simulink model "General_MPC_with_Cubic_Ls_Correction_Pose"  (R2026b)
settings: Solver=FixedStepDiscrete  StopTime=60
model workspace (MAT data in the model file):
  Velocity = 27.7777777778
  Wheel_Base = 2.866
values from neighbouring files (symbols this model uses):
  Point_Init = 0.0    [Path.sldd]
  Pose_Correction_Init = 0    [Pose_Correction.sldd]
  Pose_Init = 0.0    [MPC_Main_Dictionary.sldd]
  Reference_Path_Init = 0.0    [Path.sldd]
  Station_Calc_Init = 0.0    [Path.sldd]
  Trajectory_Init = 0.0    [Path.sldd]
  Vehicle_Cmd_Init = 0.0    [Vehicle_Controller.sldd]
libraries: simulink_extras x1
settings Model: DataDictionary=MPC_Main_Dictionary.sldd  Creator=손상민  LastModifiedBy=손상민
settings OptimizationCC: DefaultParameterBehavior=Inlined  DifferentSizesBufferReuse=on  EfficientTunableParamExpr=on  EnhancedBackFolding=on  OptimizationCustomize=off  OptimizeBlockOrder=speed  PassReuseOutputArgsAs=Individual arguments  RemoveInternalMemoryZeroInit=on  RemoveRootLevelIOMemoryZeroInit=on
settings DebuggingCC: ParameterTunabilityLossMsg=error
settings RTWCC: DataTypeReplacement=CDataTypesFixedWidth  Description=Embedded Coder  SystemTargetFile=ert.tlc  TemplateMakefile=ert_default_tmf
settings CodeAppCC: ForceParamTrailComments=on  IgnoreCustomStorageClasses=off  InsertBlockDesc=on  OperatorAnnotations=on  SFDataObjDesc=on  SimulinkDataObjDesc=on
settings ERTTargetCC: CombineSignalStateStructs=on  GenerateSampleERTMain=on  MaxIdInt16=INT16_MAX  MaxIdInt32=INT32_MAX  MaxIdInt64=INT64_MAX  MaxIdInt8=INT8_MAX  MaxIdUint16=UINT16_MAX  MaxIdUint32=UINT32_MAX  MaxIdUint64=UINT64_MAX  MaxIdUint8=UINT8_MAX  MinIdInt16=INT16_MIN  MinIdInt32=INT32_MIN  MinIdInt64=INT64_MIN  MinIdInt8=INT8_MIN

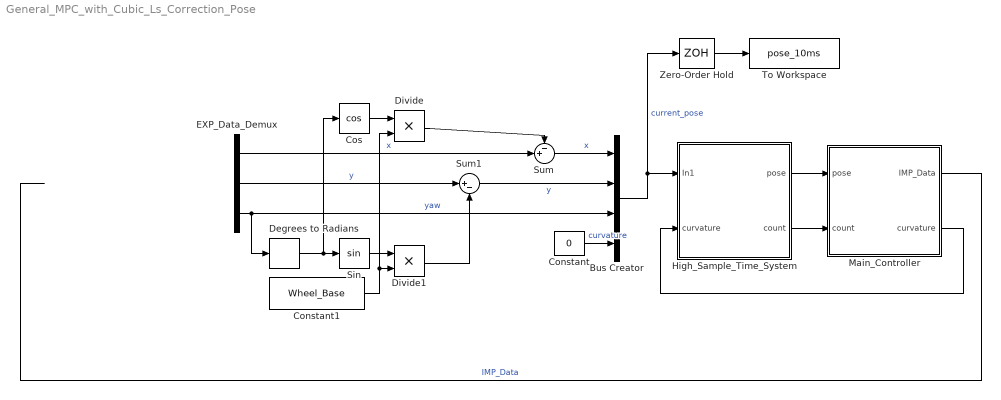
== system General_MPC_with_Cubic_Ls_Correction_Pose ==
  Bus Creator : BusCreator  Inputs=4  OutDataTypeStr=Bus: Point  NonVirtualBus=on
  Constant : Constant  Value=0
  Constant1 : Constant  Value=Wheel_Base
  Cos : Trigonometry  Operator=cos
  Degrees to Radians : simulink_extras/Transformations/Degrees to Radians
  Divide : Product  Inputs=**
  Divide1 : Product  Inputs=**
  EXP_Data_Demux : Demux  Outputs=3
  High_Sample_Time_System : Subsystem  TreatAsAtomicUnit=on  SystemSampleTime=0.1
  Main_Controller : Subsystem  TreatAsAtomicUnit=on  SystemSampleTime=0.02
  Sin : Trigonometry
  Sum : Sum  Inputs=-+|
  Sum1 : Sum  Inputs=|+-
  To Workspace : ToWorkspace  VariableName=pose_10ms  SaveFormat=Timeseries  SampleTime=-1
  Zero-Order Hold : ZeroOrderHold  SampleTime=0.01
  wires:
  Main_Controller/1(IMP_Data) -> ?  "IMP_Data"
  Zero-Order Hold/1 -> To Workspace/1
  High_Sample_Time_System/1(pose) -> Main_Controller/1(pose)
  High_Sample_Time_System/2(count) -> Main_Controller/2(count)
  EXP_Data_Demux/1 -> Sum/2  "x"
  EXP_Data_Demux/2 -> Sum1/1  "y"
  EXP_Data_Demux/3 -> Degrees to Radians/1, Bus Creator/3  "yaw"
  Constant/1 -> Bus Creator/4  "curvature"
  ? -> EXP_Data_Demux/1  "EXP_Data"
  Degrees to Radians/1 -> Cos/1, Sin/1
  Constant1/1 -> Divide/2, Divide1/2
  Cos/1 -> Divide/1
  Sin/1 -> Divide1/1
  Divide1/1 -> Sum1/2
  Sum1/1 -> Bus Creator/2  "y"
  Divide/1 -> Sum/1
  Sum/1 -> Bus Creator/1  "x"
  Bus Creator/1 -> Zero-Order Hold/1, High_Sample_Time_System/1(In1)  "current_pose"
  Main_Controller/2(curvature) -> High_Sample_Time_System/2(curvature)

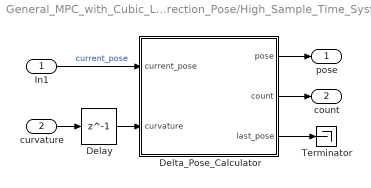
== system General_MPC_with_Cubic_Ls_Correction_Pose/High_Sample_Time_System ==
  In1 : Inport
  curvature : Inport  Port=2
  Delay : Delay  DelayLength=1  InputProcessing=Columns as channels (frame based)
  Delta_Pose_Calculator : Stateflow chart  TreatAsAtomicUnit=on
  Terminator : Terminator
  pose : Outport  OutDataTypeStr=Bus: Point
  count : Outport  Port=2  OutDataTypeStr=uint32
  wires:
  In1/1 -> Delta_Pose_Calculator/1(current_pose)  "current_pose"
  Delta_Pose_Calculator/3(last_pose) -> Terminator/1
  Delta_Pose_Calculator/2(count) -> count/1
  Delta_Pose_Calculator/1(pose) -> pose/1
  curvature/1 -> Delay/1
  Delay/1 -> Delta_Pose_Calculator/2(curvature)

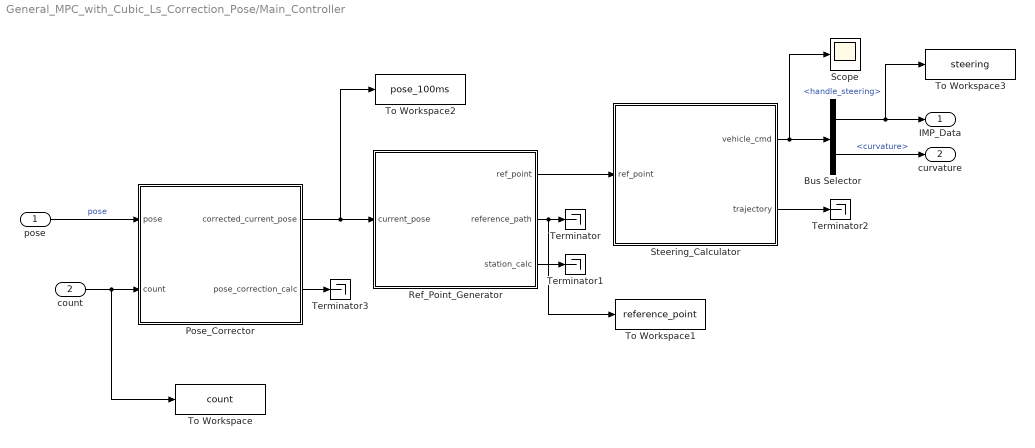
== system General_MPC_with_Cubic_Ls_Correction_Pose/Main_Controller ==
  pose : Inport  OutDataTypeStr=Bus: Point
  count : Inport  Port=2  OutDataTypeStr=uint32
  Bus Selector : BusSelector  OutputSignals=handle_steering,curvature
  Pose_Corrector : Stateflow chart  TreatAsAtomicUnit=on
  Ref_Point_Generator : Stateflow chart  TreatAsAtomicUnit=on
  Scope : Scope
      settings: ActiveDisplayYMinimum=-65.96053155183364  ActiveDisplayYMaximum=44.846225949844211
  Steering_Calculator : Stateflow chart  TreatAsAtomicUnit=on
  Terminator{,1..3} (4 alike) : Terminator
  To Workspace : ToWorkspace  VariableName=count  SaveFormat=Timeseries  SampleTime=-1
  To Workspace1 : ToWorkspace  VariableName=reference_point  SaveFormat=Timeseries  SampleTime=-1
  To Workspace2 : ToWorkspace  VariableName=pose_100ms  SaveFormat=Timeseries  SampleTime=-1
  To Workspace3 : ToWorkspace  VariableName=steering  SaveFormat=Timeseries  SampleTime=-1
  IMP_Data : Outport
  curvature : Outport  Port=2
  wires:
  pose/1 -> Pose_Corrector/1(pose)  "pose"
  Ref_Point_Generator/2(reference_path) -> To Workspace1/1, Terminator/1
  Ref_Point_Generator/1(ref_point) -> Steering_Calculator/1(ref_point)
  Steering_Calculator/1(vehicle_cmd) -> Scope/1, Bus Selector/1
  Ref_Point_Generator/3(station_calc) -> Terminator1/1
  Bus Selector/1 -> To Workspace3/1, IMP_Data/1  "<handle_steering>"
  Bus Selector/2 -> curvature/1  "<curvature>"
  Steering_Calculator/2(trajectory) -> Terminator2/1
  Pose_Corrector/1(corrected_current_pose) -> To Workspace2/1, Ref_Point_Generator/1(current_pose)
  count/1 -> To Workspace/1, Pose_Corrector/2(count)
  Pose_Corrector/2(pose_correction_calc) -> Terminator3/1

== matlab function General_MPC_with_Cubic_Ls_Correction_Pose/Main_Controller/Steering_Calculator ==
  data: out_para function_output Bus: Point size=201; out_para function_output Bus: Vehicle_Cmd size=1; out_para function_output double size=1; ref_point input Bus: Point size=1; vehicle_cmd output Bus: Vehicle_Cmd size=1 =Vehicle_Cmd_Init; trajectory output Bus: Point size=201 =Trajectory_Init
function out_para = Generate_Trajectory

out_para = trajectory;

sampleTime = 0.1;
wheelbase = 2.866;
velocity = 30/3.6;
steering = deg2rad(vehicle_cmd.steering);

predictionHorizon = 15;

xTarget = ref_point.x;
yTarget = ref_point.y;
headingTarget = wrap_to_pi_local(ref_point.yaw);
curvatureTarget = ref_point.curvature;

heading0 = 0.0;
curvature0 = tan(steering) / wheelbase;

pointSpacing = sampleTime * abs(velocity);
pointCount = predictionHorizon + 1;

chordLength = hypot(xTarget, yTarget);

if chordLength <= 1.0e-6 || pointSpacing <= 1.0e-12
    for i = 1:pointCount
        out_para(i).x = 0.0;
        out_para(i).y = 0.0;
        out_para(i).yaw = 0.0;
        out_para(i).curvature = curvature0;
    end
    return
end

tangent0 = [cos(heading0), sin(heading0)];
tangent1 = [cos(headingTarget), sin(headingTarget)];

normal0 = [-sin(heading0), cos(heading0)];
normal1 = [-sin(headingTarget), cos(headingTarget)];

velocity0 = chordLength * tangent0;
velocity1 = chordLength * tangent1;

acceleration0 = chordLength^2 * curvature0 * normal0;
acceleration1 = chordLength^2 * curvatureTarget * normal1;

boundaryMatrix = [ ...
    1, 0, 0,  0,  0,  0;
    0, 1, 0,  0,  0,  0;
    0, 0, 2,  0,  0,  0;
    1, 1, 1,  1,  1,  1;
    0, 1, 2,  3,  4,  5;
    0, 0, 2,  6, 12, 20];

boundaryValues = [ ...
    0.0, 0.0;
    velocity0;
    acceleration0;
    xTarget, yTarget;
    velocity1;
    acceleration1];

coeff = boundaryMatrix \ boundaryValues;

denseCount = 10001;
uDense = linspace(0.0, 1.0, denseCount).';

[denseX, denseY, ~, ~, ~, ~] = ...
    evaluate_polynomial(coeff, uDense);

denseArc = [0.0; cumsum(hypot(diff(denseX), diff(denseY)))];
totalLength = denseArc(end);

requestedArc = (0:predictionHorizon).' * pointSpacing;
requestedArc = min(requestedArc, totalLength);

u = invert_arc_length(denseArc, uDense, requestedArc);

[x, y, dx, dy, ddx, ddy] = ...
    evaluate_polynomial(coeff, u);

speedSquared = dx.^2 + dy.^2;
speedSquared = max(speedSquared, 1.0e-12);

yaw = atan2(dy, dx);

curvature = ...
    (dx .* ddy - dy .* ddx) ./ ...
    (speedSquared .^ 1.5);

for i = 1:pointCount
    out_para(i).x = x(i);
    out_para(i).y = y(i);
    out_para(i).yaw = yaw(i);
    out_para(i).curvature = curvature(i);
end

end


function uQuery = invert_arc_length(arcValues, uValues, queryValues)

queryCount = numel(queryValues);
arcCount = numel(arcValues);

uQuery = zeros(queryCount, 1);

searchIndex = 1;

for i = 1:queryCount

    queryArc = queryValues(i);

    if queryArc <= arcValues(1)

        uQuery(i) = uValues(1);

    elseif queryArc >= arcValues(arcCount)

        uQuery(i) = uValues(arcCount);

    else

        while searchIndex < arcCount && ...
                arcValues(searchIndex + 1) < queryArc

            searchIndex = searchIndex + 1;

        end

        lowerIndex = searchIndex;
        upperIndex = lowerIndex + 1;

        while upperIndex <= arcCount && ...
                arcValues(upperIndex) <= arcValues(lowerIndex)

            upperIndex = upperIndex + 1;

        end

        if upperIndex > arcCount

            uQuery(i) = uValues(lowerIndex);

        else

            arcInterval = ...
                arcValues(upperIndex) - arcValues(lowerIndex);

            ratio = ...
                (queryArc - arcValues(lowerIndex)) / arcInterval;

            ratio = min(max(ratio, 0.0), 1.0);

            uQuery(i) = ...
                uValues(lowerIndex) + ...
                ratio * (uValues(upperIndex) - uValues(lowerIndex));

        end
    end
end

end


function [x, y, dx, dy, ddx, ddy] = evaluate_polynomial(coeff, u)

basis0 = [ ...
    ones(size(u)), ...
    u, ...
    u.^2, ...
    u.^3, ...
    u.^4, ...
    u.^5];

basis1 = [ ...
    zeros(size(u)), ...
    ones(size(u)), ...
    2*u, ...
    3*u.^2, ...
    4*u.^3, ...
    5*u.^4];

basis2 = [ ...
    zeros(size(u)), ...
    zeros(size(u)), ...
    2*ones(size(u)), ...
    6*u, ...
    12*u.^2, ...
    20*u.^3];

position = basis0 * coeff;
firstDerivative = basis1 * coeff;
secondDerivative = basis2 * coeff;

x = position(:, 1);
y = position(:, 2);

dx = firstDerivative(:, 1);
dy = firstDerivative(:, 2);

ddx = secondDerivative(:, 1);
ddy = secondDerivative(:, 2);

end


function angle = wrap_to_pi_local(angle)

angle = mod(angle + pi, 2*pi) - pi;

end

== matlab function General_MPC_with_Cubic_Ls_Correction_Pose/Main_Controller/Steering_Calculator ==
function out_para = MPC

out_para = vehicle_cmd;

sampleTime = 0.1;
wheelbase = 2.866;

predictionHorizon = double(15);
controlHorizon = double(10);

wheelSteering = deg2rad(vehicle_cmd.steering);
targetSpeed = 30/3.6;

traj = zeros(4, predictionHorizon + 1);

for index = 1:predictionHorizon + 1
    traj(1,index) = trajectory(index).x;
    traj(2,index) = trajectory(index).y;
    traj(3,index) = trajectory(index).yaw;
    traj(4,index) = trajectory(index).curvature;
end

R = 500 * eye(controlHorizon);
F = 200 * eye(controlHorizon);
Q = kron(eye(predictionHorizon), diag([100 500 500]));

steerMax = deg2rad(35);
duMax = deg2rad(5);

W = tril(ones(controlHorizon));

Aineq = [W; -W];

bineq = [ ...
    steerMax * ones(controlHorizon,1) - wheelSteering;
    steerMax * ones(controlHorizon,1) + wheelSteering];

A_k = [ ...
    1 0 -targetSpeed * sin(traj(3,2)) * sampleTime;
    0 1  targetSpeed * cos(traj(3,2)) * sampleTime;
    0 0  1];

B_k = [ ...
    0;
    0;
    targetSpeed * sampleTime / wheelbase];

Abar_k = zeros(4);
Abar_k(1:3,1:3) = A_k;
Abar_k(1:3,4) = B_k;
Abar_k(4,4) = 1;

Bbar_k = [B_k; 1];

cbar = [eye(3), zeros(3,1)];

Psi_k = zeros(3 * predictionHorizon, 4);

for row = 1:predictionHorizon
    Psi_k(3*row-2:3*row,:) = ...
        cbar * (Abar_k^row);
end

Theta_k = zeros(3 * predictionHorizon, controlHorizon);

for row = 1:predictionHorizon
    for col = 1:controlHorizon

        powerValue = row - col;

        if powerValue >= 0
            Theta_k(3*row-2:3*row,col) = ...
                cbar * (Abar_k^powerValue) * Bbar_k;
        end

    end
end

Pi_k = zeros(3 * predictionHorizon, 4 * predictionHorizon);

for row = 1:predictionHorizon
    for col = 1:predictionHorizon

        powerValue = row - col;

        if powerValue >= 0
            Pi_k(3*row-2:3*row,4*col-3:4*col) = ...
                cbar * (Abar_k^powerValue);
        end

    end
end

steeringRef = atan(wheelbase * traj(4,:));

X_ref = [ ...
    traj(1:3,:);
    steeringRef];

G_k = zeros(4 * predictionHorizon, 1);

for row = 1:predictionHorizon

    duRef = steeringRef(row+1) - steeringRef(row);

    G_k(4*row-3:4*row) = ...
        X_ref(:,row+1) ...
        - Abar_k * X_ref(:,row) ...
        - Bbar_k * duRef;

end

Y_ref = reshape( ...
    traj(1:3,2:predictionHorizon+1), ...
    [], 1);

X0 = [ ...
    traj(1:3,1);
    wheelSteering];

E_k = ...
    Psi_k * X0 ...
    + Pi_k * G_k ...
    - Y_ref;

U_ref = steeringRef(2:controlHorizon+1).';

EU_k = ...
    ones(controlHorizon,1) * wheelSteering ...
    - U_ref;

S_k = ...
    2 * E_k.' * Q * Theta_k ...
    + 2 * EU_k.' * F * W;

H_k = 2 * ( ...
    Theta_k.' * Q * Theta_k ...
    + R ...
    + W.' * F * W);

H_k = 0.5 * (H_k + H_k.');

options = optimoptions( ...
    'quadprog', ...
    'Algorithm', 'active-set', ...
    'Display', 'off');

lb = -duMax * ones(controlHorizon,1);
ub =  duMax * ones(controlHorizon,1);

x0 = zeros(controlHorizon,1);

dU = quadprog( ...
    H_k, ...
    S_k.', ...
    Aineq, ...
    bineq, ...
    [], ...
    [], ...
    lb, ...
    ub, ...
    x0, ...
    options);

if isempty(dU)
    outWheelSteering = wheelSteering;
else
    outWheelSteering = wheelSteering + dU(1);
end

out_para.steering = rad2deg(outWheelSteering);
out_para.curvature = tan(outWheelSteering) / wheelbase;

end

== matlab function General_MPC_with_Cubic_Ls_Correction_Pose/Main_Controller/Steering_Calculator ==
function out_para = Calc_Handle_Steering

equivalentSteerDeg = [ ...
    -38.0000000015 -37.5537097659 -37.1100763419 -36.6690267064 -36.2304905472 -35.7944001026 ...
    -35.3606900619 -34.9292974092 -34.5001613191 -34.0732230402 -33.6484257893 -33.2257146793 ...
    -32.8050365911 -32.3863401170 -31.9695754559 -31.5546943618 -31.1416500661 -30.7303971963 ...
    -30.3208917313 -29.9130909189 -29.5069532444 -29.1024383621 -28.6995070462 -28.2981211430 ...
    -27.8982435354 -27.4998380812 -27.1028695774 -26.7073037505 -26.3131071606 -25.9202472249 ...
    -25.5286921549 -25.1384109184 -24.7493732347 -24.3615495211 -23.9749108816 -23.5894290638 ...
    -23.2050764567 -22.8218260419 -22.4396513910 -22.0585266399 -21.6784264440 -21.2993259988 ...
    -20.9212009824 -20.5440275610 -20.1677823626 -19.7924424606 -19.4179853631 -19.0443889805 ...
    -18.6716316310 -18.2996920094 -17.9285491937 -17.5581826079 -17.1885720119 -16.8196975175 ...
    -16.4515395418 -16.0840788091 -15.7172963351 -15.3511734516 -14.9856917222 -14.6208329945 ...
    -14.2565793874 -13.8929132418 -13.5298171372 -13.1672739009 -12.8052665504 -12.4437783367 ...
    -12.0827926977 -11.7222932796 -11.3622638965 -11.0026885634 -10.6435514521 -10.2848369165 ...
    -9.9265294385 -9.5686136760 -9.2110744293 -8.8538966284 -8.4970653414 -8.1405657596 ...
    -7.7843831967 -7.4285030781 -7.0729109402 -6.7175924190 -6.3625332509 -6.0077192620 ...
    -5.6531363648 -5.2987705549 -4.9446079016 -4.5906345476 -4.2368366983 -3.8832006231 ...
    -3.5297126453 -3.1763591407 -2.8231265306 -2.4700012785 -2.1169698838 -1.7640188790 ...
    -1.4111348234 -1.0583043010 -0.7055139116 -0.3527502699 0.0000000000 0.3527502699 ...
    0.7055139116 1.0583043010 1.4111348234 1.7640188790 2.1169698838 2.4700012785 ...
    2.8231265306 3.1763591407 3.5297126453 3.8832006231 4.2368366983 4.5906345476 ...
    4.9446079016 5.2987705549 5.6531363648 6.0077192620 6.3625332509 6.7175924190 ...
    7.0729109402 7.4285030781 7.7843831967 8.1405657596 8.4970653414 8.8538966284 ...
    9.2110744293 9.5686136760 9.9265294385 10.2848369165 10.6435514521 11.0026885634 ...
    11.3622638965 11.7222932796 12.0827926977 12.4437783367 12.8052665504 13.1672739009 ...
    13.5298171372 13.8929132418 14.2565793874 14.6208329945 14.9856917222 15.3511734516 ...
    15.7172963351 16.0840788091 16.4515395418 16.8196975175 17.1885720119 17.5581826079 ...
    17.9285491937 18.2996920094 18.6716316310 19.0443889805 19.4179853631 19.7924424606 ...
    20.1677823626 20.5440275610 20.9212009824 21.2993259988 21.6784264440 22.0585266399 ...
    22.4396513910 22.8218260419 23.2050764567 23.5894290638 23.9749108816 24.3615495211 ...
    24.7493732347 25.1384109184 25.5286921549 25.9202472249 26.3131071606 26.7073037505 ...
    27.1028695774 27.4998380812 27.8982435354 28.2981211430 28.6995070462 29.1024383621 ...
    29.5069532444 29.9130909189 30.3208917313 30.7303971963 31.1416500661 31.5546943618 ...
    31.9695754559 32.3863401170 32.8050365911 33.2257146793 33.6484257893 34.0732230402 ...
    34.5001613191 34.9292974092 35.3606900619 35.7944001026 36.2304905472 36.6690267064 ...
    37.1100763419 37.5537097659 38.0000000015
    ].';

rackMap = (-90.0:0.9:90.0).';

wheelSteeringDeg = vehicle_cmd.steering;

rackDisplacement = interp1(equivalentSteerDeg, rackMap, wheelSteeringDeg, 'linear');
out_para = rackDisplacement * 360.0 / 56.25;

end

== matlab function General_MPC_with_Cubic_Ls_Correction_Pose/High_Sample_Time_System/Delta_Pose_Calculator ==
  data: out_para function_output; pose output Bus: Point size=5 =Pose_Init; current_pose input Bus: Point size=1; count output uint32 size=1 =0; last_pose output Bus: Point size=1 =Point_Init; curvature input double size=1
function out_para = Calc_Delta_Pose 

out_para = pose;

index = mod(count,5) + 1;

out_para(index) = current_pose;
out_para(index).curvature = curvature;

== matlab function General_MPC_with_Cubic_Ls_Correction_Pose/Main_Controller/Ref_Point_Generator ==
  data: out_para function_output Bus: Reference_Path size=1; out_para function_output Bus: Station_Calc size=1; out_para function_output Bus: Point size=1; ref_point output Bus: Point size=1 =Point_Init; reference_path output Bus: Reference_Path size=1 =Reference_Path_Init; current_pose input Bus: Point size=1; station_calc output Bus: Station_Calc size=1 =Station_Calc_Init
function out_para = Map_Generator 

out_para = reference_path;

ds = 0.1;

x_data = [70 75 80 85 90 95 100 105 110 115 120 125 130 135 140 145];
y_data = [0 0.2 1.1 2.4 3.3 3.5 3.5 3.5 3.5 3.5 3.5 3.3 2.4 1.1 0.2 0];

pp = spline(x_data, [0 y_data 0]);

x_temp = linspace(0, 500, 10000);
y_temp = zeros(size(x_temp));

idx = (x_temp >= 70) & (x_temp <= 145);
y_temp(idx) = ppval(pp, x_temp(idx));

s_temp = [0 cumsum(hypot(diff(x_temp), diff(y_temp)))];

station = 0:ds:5007;

x = interp1(s_temp, x_temp, station, 'pchip');
y = interp1(s_temp, y_temp, station, 'pchip');

dx_ds = gradient(x, station);
dy_ds = gradient(y, station);

yaw = unwrap(atan2(dy_ds, dx_ds));

ddx_ds2 = gradient(dx_ds, station);
ddy_ds2 = gradient(dy_ds, station);

curvature = (dx_ds .* ddy_ds2 - dy_ds .* ddx_ds2) ./ ...
    (dx_ds.^2 + dy_ds.^2).^(3/2);

N = length(x);

for i = 1:N
    out_para.points(i).x = x(i);
    out_para.points(i).y = y(i);
    out_para.points(i).yaw = yaw(i);
    out_para.points(i).curvature = curvature(i);
end

out_para.length = uint32(N);

== matlab function General_MPC_with_Cubic_Ls_Correction_Pose/Main_Controller/Ref_Point_Generator ==
function out_para = Calc_Station 

out_para = station_calc;

min_dist = inf;
start_idx = double(out_para.station_index);

if out_para.predictive_length == 0

    % initialize
    for i = 1:reference_path.length
        dx = reference_path.points(i).x - current_pose.x;
        dy = reference_path.points(i).y - current_pose.y;

        dist = dx * dx + dy * dy;

        if dist < min_dist
            min_dist = dist;
            out_para.station_index = uint32(i);
        end
    end

else

    for i = 1:out_para.predictive_length
        dx = out_para.predictive_station(i).x - current_pose.x;
        dy = out_para.predictive_station(i).y - current_pose.y;

        dist = dx * dx + dy * dy;

        if dist < min_dist
            min_dist = dist;
            out_para.station_index = uint32(start_idx + i - 1);
        end
    end

end

N_ref = double(reference_path.length);
start_idx = double(out_para.station_index);

N_pred = min(50, N_ref - start_idx + 1);

for i = 1:N_pred
    idx = start_idx + i - 1;

    out_para.predictive_station(i).x = reference_path.points(idx).x;
    out_para.predictive_station(i).y = reference_path.points(idx).y;
    out_para.predictive_station(i).yaw = reference_path.points(idx).yaw;
    out_para.predictive_station(i).curvature = reference_path.points(idx).curvature;
end

out_para.predictive_length = uint32(N_pred);

== matlab function General_MPC_with_Cubic_Ls_Correction_Pose/Main_Controller/Ref_Point_Generator ==
function out_para = Calc_Ref_Point 

out_para = ref_point;

ds = 0.1;
velocity = 30/3.6;
preview_second = 1.5;
 
preview_distance = velocity * preview_second;

preview_index = double(station_calc.station_index) + round(preview_distance / ds);
preview_index = min(preview_index, double(reference_path.length));

ref = reference_path.points(preview_index);

dx = ref.x - current_pose.x;
dy = ref.y - current_pose.y;

yaw = deg2rad(current_pose.yaw);
c = cos(yaw);
s = sin(yaw);

out_para.x =  c * dx + s * dy;
out_para.y = -s * dx + c * dy;
out_para.yaw = atan2(sin(ref.yaw - yaw), cos(ref.yaw - yaw));

out_para.curvature = ref.curvature;

== stateflow chart General_MPC_with_Cubic_Ls_Correction_Pose/Main_Controller/Pose_Corrector ==
  (default) -> (junction 4)
  (junction 4) -> (junction 7) [order 1] : [Is_Changed]
  (junction 4) -> (junction 13) [order 2] : {
      | pose_correction_calc = Update_Pose_Correction;
      | }
  (junction 7) -> (junction 15) : {
      | pose_correction_calc = Calc_Pose_Correction;
      | }
  (junction 15) -> (junction 13)
  (junction 13) -> (junction 18) : {
      | corrected_current_pose = Calc_Current_Pose;
      | }
  data: out function_output; out_para function_output; out_para function_output; out_para function_output; pose input Bus: Point size=5; corrected_current_pose output Bus: Point size=1 =Point_Init; count input uint32 size=1; pose_correction_calc output Bus: Pose_Correction_Calc size=1 =Pose_Correction_Init
  function out = Is_Changed:
    | function out = Is_Changed 
    | 
    | out = pose_correction_calc.last_count ~= count;
  function out_para = Calc_Pose_Correction:
    | function out_para = Calc_Pose_Correction
    | % Stateflow/MATLAB chart shared data: pose, count, pose_correction_calc.
    | % pose(i).x, pose(i).y: world coordinates [m]; pose(i).yaw: [deg].
    | % pose is a FIVE-SLOT CIRCULAR BUFFER. Current slot = mod(count,5)+1.
    | % count increments once per new pose. Do not divide count by five.
    | % Call after writing a new sensor pose and advancing its count.
    | % Output is POSITIVE movement for current_pose + correction_value.
    | % Five past/current poses predict next-100-ms movement; add that movement.
    | % Six points are uniform in current-heading x, as in the earlier comparison.
    | % Deliberate XY bias toward the previous linear correction; yaw stays cubic LS.
    | % outward_mix=0: current LS; 1: old linear XY. Halfway is an A/B candidate,
    | % not a closed-loop optimum and not a guarantee about unknown future actual.
    | 
    | 
    | outward_mix = 0.0; % Try 0.25, 0.5, 1 in separate closed-loop runs.
    | assert(outward_mix >= 0 && outward_mix <= 1);
    | 
    | out_para = pose_correction_calc;
    | out_para.inner_count = uint8(1);
    | out_para.last_count = count;
    | 
    | count_value = double(count);
    | assert(isfinite(count_value) && count_value >= 0 && count_value == floor(count_value));
    | assert(numel(pose) >= 5);
    | idx = mod(count_value, 5) + 1;
    | previous_idx = mod(count_value - 1, 5) + 1;
    | 
    | % First recorded pose count is 1 in the supplied simulation data.
    | % Set this to 0 if your first valid pose is written at count=0.
    | first_pose_count = 1;
    | available_poses = max(0, count_value - first_pose_count + 1);
    | 
    | num_points = 6;
    | alpha = (0:5) / 5;
    | x_sample = zeros(1, 6);
    | y_sample = zeros(1, 6);
    | yaw_sample = zeros(1, 6);
    | step_x = 0;
    | step_y = 0;
    | 
    | %% 1. Startup / degenerate-geometry fallback: original linear correction
    | if available_poses >= 2
    |     step_x = double(pose(idx).x) - double(pose(previous_idx).x);
    |     step_y = double(pose(idx).y) - double(pose(previous_idx).y);
    |     step_yaw = double(pose(idx).yaw) - double(pose(previous_idx).yaw);
    |     wrapped_step_yaw = mod(step_yaw + 180, 360) - 180;
    | 
    |     x_sample = alpha * step_x;
    |     y_sample = alpha * step_y;
    |     if hypot(step_x, step_y) > 1e-9
    |         yaw_sample = alpha * wrapped_step_yaw;
    |     else
    |         % Preserve the original in-place rotation treatment.
    |         smooth_alpha = 3 * alpha.^2 - 2 * alpha.^3;
    |         yaw_sample = smooth_alpha * wrapped_step_yaw;
    |     end
    | end
    | 
    | %% 2. Five-pose cubic least squares, anchored at current pose
    | if available_poses >= 5
    |     origin_x = double(pose(idx).x);
    |     origin_y = double(pose(idx).y);
    |     current_yaw = double(pose(idx).yaw) * pi / 180;
    |     c = cos(current_yaw);
    |     s = sin(current_yaw);
    | 
    |     local_x = zeros(5, 1);
    |     local_y = zeros(5, 1);
    |     yaw_history = zeros(5, 1);
    |     for h = 1:5
    |         % Chronological K-4,...,K, regardless of current buffer slot.
    |         history_idx = mod(count_value - 5 + h, 5) + 1;
    |         relative_x = double(pose(history_idx).x) - origin_x;
    |         relative_y = double(pose(history_idx).y) - origin_y;
    |         local_x(h) = c * relative_x + s * relative_y;
    |         local_y(h) = -s * relative_x + c * relative_y;
    |         yaw_history(h) = double(pose(history_idx).yaw);
    |     end
    | 
    |     % Unwrap backwards from current physical yaw. Current relative yaw = 0.
    |     relative_yaw = zeros(5, 1);
    |     for h = 4:-1:1
    |         yaw_increment = yaw_history(h + 1) - yaw_history(h);
    |         yaw_increment = mod(yaw_increment + 180, 360) - 180;
    |         relative_yaw(h) = relative_yaw(h + 1) - yaw_increment;
    |     end
    | 
    |     L = c * step_x + s * step_y;
    |     valid_history = L > 1e-8;
    |     for h = 2:5
    |         if local_x(h) - local_x(h - 1) <= 1e-9
    |             valid_history = false;
    |         end
    |     end
    |     if ~all(isfinite(local_x)) || ~all(isfinite(local_y)) || ...
    |             ~all(isfinite(relative_yaw))
    |         valid_history = false;
    |     end
    | 
    |     if valid_history
    |         % f(u)=a1*u+a2*u^2+a3*u^3; omit constant so f(0)=0 exactly.
    |         % Four previous observations, three coefficients. All sizes fixed.
    |         A = zeros(4, 3);
    |         B = zeros(4, 2); % Columns: local Y and recorded physical yaw change.
    |         for h = 1:4
    |             z = local_x(h) / L;
    |             A(h, 1) = z;
    |             A(h, 2) = z * z;
    |             A(h, 3) = z * z * z;
    |             B(h, 1) = local_y(h);
    |             B(h, 2) = relative_yaw(h);
    |         end
    | 
    |         % QR least squares; avoid normal equations A'*A.
    |         [Q, R] = qr(A, 0);
    |         if rcond(R) > 1e-10
    |             coefficients = R \ (Q.' * B);
    |             for i = 1:num_points
    |                 u = alpha(i);
    |                 u2 = u * u;
    |                 u3 = u2 * u;
    |                 forward_x = L * u;
    |                 forward_y_ls = coefficients(1, 1) * u + ...
    |                     coefficients(2, 1) * u2 + coefficients(3, 1) * u3;
    |                 % Both curves share forward_x=L*u. Move only local Y.
    |                 previous_local_y = -s * step_x + c * step_y;
    |                 forward_y_linear = previous_local_y * u;
    |                 forward_y = forward_y_ls + ...
    |                     outward_mix * (forward_y_linear - forward_y_ls);
    |                 forward_yaw = coefficients(1, 2) * u + ...
    |                     coefficients(2, 2) * u2 + coefficients(3, 2) * u3;
    | 
    |                 % Rotate to WORLD axes for additive forward correction.
    |                 x_sample(i) = c * forward_x - s * forward_y;
    |                 y_sample(i) = s * forward_x + c * forward_y;
    |                 yaw_sample(i) = mod(forward_yaw + 180, 360) - 180;
    |             end
    |         end
    |     end
    | end
    | 
    | %% 3. Keep the existing output bus / structure
    | for i = 1:num_points
    |     out_para.correction_value(i).x = x_sample(i);
    |     out_para.correction_value(i).y = y_sample(i);
    |     out_para.correction_value(i).yaw = yaw_sample(i);
    | end
    | 
    | end
  function out_para = Update_Pose_Correction:
    | function out_para = Update_Pose_Correction 
    | 
    | out_para = pose_correction_calc;
    | 
    | if out_para.inner_count < uint8(11)
    |     out_para.inner_count = out_para.inner_count + uint8(1);
    | end
  function out_para = Calc_Current_Pose:
    | function out_para = Calc_Current_Pose 
    | 
    | out_para = corrected_current_pose;
    | 
    | 
    | index = mod(count,5) + 1;
    | 
    | idx = pose_correction_calc.inner_count;
    | correction_value = pose_correction_calc.correction_value(idx);
    | 
    | out_para.x = pose(index).x + correction_value.x;
    | out_para.y = pose(index).y + correction_value.y;
    | out_para.yaw = pose(index).yaw + correction_value.yaw;
    | out_para.curvature = pose(index).curvature;
